simulink model "FULL_CAR_SIM"  (R2025b)
settings: Solver=FixedStepAuto  StartTime=0.0  StopTime=5  FixedStep=dT  RelTol=1e-3
values from neighbouring files (symbols this model uses):
  fc = 50    [FULL_CAR_MODEL.m]
  Fuzzy_Gain = 2300    [FULL_CAR_MODEL.m]
  Kd = 2873    [FULL_CAR_MODEL.m]
  Ki = 250000    [FULL_CAR_MODEL.m]
  Kp = 23750    [FULL_CAR_MODEL.m]
  l1 = 1.2    [FULL_CAR_MODEL.m]
  w1 = 0.7    [FULL_CAR_MODEL.m]
libraries: fuzblock x4, slpidlib x4, simulink x1
settings Model: Creator=andorian  LastModifiedBy=andac

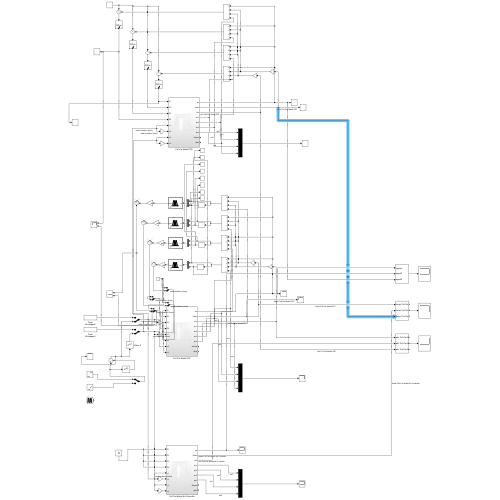
[thumbnail: Simulink's stored preview of the top-level diagram]
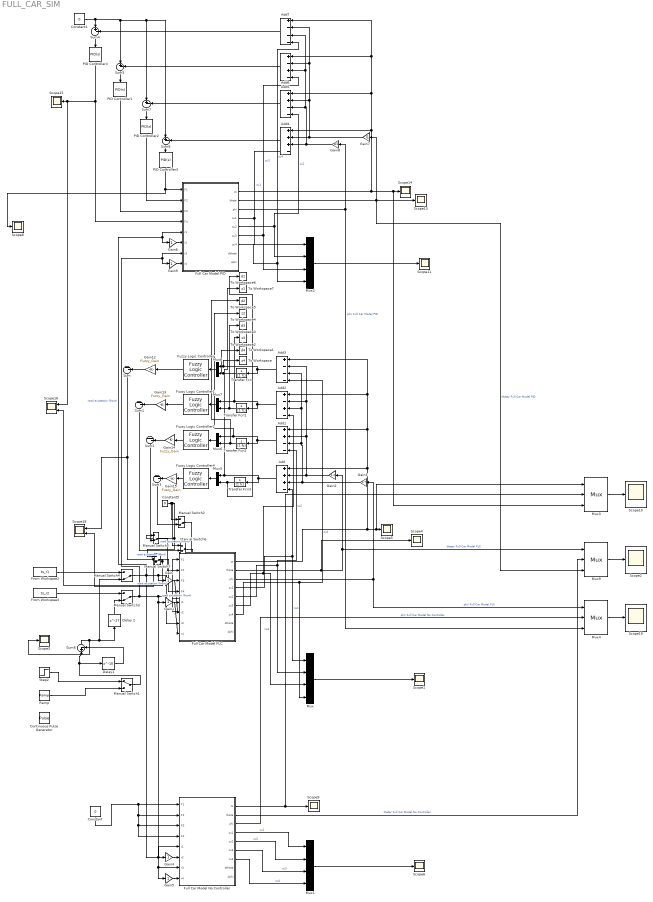
== system FULL_CAR_SIM ==
  Add : Sum  Inputs=+++-
  Add1 : Sum  Inputs=++--
  Add2 : Sum  Inputs=+-+-
  Add3 : Sum  Inputs=+---
  Add4 : Sum  Inputs=+++-
  Add5 : Sum  Inputs=++--
  Add6 : Sum  Inputs=+-+-
  Add7 : Sum  Inputs=+---
  Constant : Constant  Value=0
  Constant1 : Constant  Value=0
  Constant5 : Constant  Value=0
  Continuous Pulse Generator : DiscretePulseGenerator  PulseType=Time based  Period=0.5  PulseWidth=50
  Delay 2 : Delay  DelayLength=27
  Delay1 : Delay  DelayLength=10
  From Workspae2 : FromWorkspace  VariableName=ts_r1
  From Workspae3 : FromWorkspace  VariableName=ts_r2
  Full Car Model FLC : Subsystem
  Full Car Model No Controller : Subsystem
  Full Car Model PID : Subsystem
  Fuzzy Logic Controller{,1..2,4} (4 alike) : fuzblock/Fuzzy Logic  Controller  FIS=susp_fis_cont  OutputSampleNumber=101  DataType=double  UseLookupTable=off  NumBreakpoints=10  FuzzifiedInputs=off  RuleFiringStrengths=off  RuleOutputs=off  AggregatedOutputs=off  SimulateUsing=Interpreted execution  OutOfRangeInputValueMessage=warning  NoRuleFiredMessage=warning  EmptyOutputFuzzySetMessage=warning
  Gain{,1,4..6,9} (6 alike) : Gain
  Gain{12..15} (4 alike) : Gain  Gain=Fuzzy_Gain
  Gain2 : Gain  Gain=1.2
  Gain3 : Gain  Gain=0.7
  Gain7 : Gain  Gain=l1
  Gain8 : Gain  Gain=w1
  Manual Switch1 : ManualSwitch
  Manual Switch{2..7} (6 alike) : ManualSwitch  CurrentSetting=0
  Mux : Mux
  Mux1 : Mux
  Mux2 : Mux
  Mux3 : Mux  Inputs=3
      settings: DisplayOption=signals
  Mux4 : Mux  Inputs=3
      settings: DisplayOption=signals
  Mux{5..8} (4 alike) : Mux  Inputs=2
  Mux9 : Mux  Inputs=3
      settings: DisplayOption=signals
  PID Controller1 : slpidlib/PID Controller  Controller=PID  Form=Parallel  TimeDomain=Continuous-time  UseExternalTs=off  SampleTime=-1  IntegratorMethod=Forward Euler  FilterMethod=Forward Euler  ControllerParametersSource=internal  P=Kp  I=Ki  UseKiTs=off  D=Kd  UseExternalDerivativeSource=off  N=57.4302728612139  UseFilter=on  TunerSelectOption=Transfer Function Based (PID Tuner App)  InitialConditionSource=internal  InitialConditionForIntegrator=0  InitialConditionForFilter=0  DifferentiatorICPrevScaledInput=0  ExternalReset=none  TrackingMode=off  Kt=1  LimitOutput=on  SatLimitsSource=internal  UpperSaturationLimit=2000  LowerSaturationLimit=-2000  LinearizeAsGain=on  AntiWindupMode=back-calculation  Kb=1  LimitIntegrator=off  UpperIntegratorSaturationLimit=inf  LowerIntegratorSaturationLimit=-inf  POutMin=[]  POutMax=[]  IOutMin=[]  IOutMax=[]  DOutMin=[]  DOutMax=[]  NOutMin=[]  NOutMax=[]  SumOutMin=[]  SumOutMax=[]  SaturationOutMin=[]  SaturationOutMax=[]  PParamMin=[]  PParamMax=[]  IParamMin=[]  IParamMax=[]  DParamMin=[]  DParamMax=[]  NParamMin=[]  NParamMax=[]  KbParamMin=[]  KbParamMax=[]  KtParamMin=[]  KtParamMax=[]  KbOutMin=[]  KbOutMax=[]  KtOutMin=[]  KtOutMax=[]  IntegratorOutMin=[]  IntegratorOutMax=[]  FilterOutMin=[]  FilterOutMax=[]  SumI1OutMin=[]  SumI1OutMax=[]  SumI2OutMin=[]  SumI2OutMax=[]  SumI3OutMin=[]  SumI3OutMax=[]  SumI4OutMin=[]  SumI4OutMax=[]  SumDOutMin=[]  SumDOutMax=[]  DifferentiatorOutMin=[]  DifferentiatorOutMax=[]  FilterDiffOutCoefMin=[]  FilterDiffOutCoefMax=[]  ReciprocalOutMin=[]  ReciprocalOutMax=[]  SumDenOutMin=[]  SumDenOutMax=[]  SumNumOutMin=[]  SumNumOutMax=[]  DivideOutMin=[]  DivideOutMax=[]  UdiffTsProdOutMin=[]  UdiffTsProdOutMax=[]  NTsProdOutMin=[]  NTsProdOutMax=[]  UintegralTsProdOutMin=[]  UintegralTsProdOutMax=[]  UngainTsProdOutMin=[]  UngainTsProdOutMax=[]  ClampingZeroOutDataTypeStr=Inherit: Inherit via back propagation  ClampingZeroOutMin=[]  ClampingZeroOutMax=[]  FilterDenConstantOutDataTypeStr=Inherit: Inherit via back propagation  FilterDenConstantOutMin=[]  FilterDenConstantOutMax=[]  PCopyOutDataTypeStr=Inherit: Inherit via back propagation  PCopyOutMin=[]  PCopyOutMax=[]  NCopyOutDataTypeStr=Inherit: Inherit via back propagation  NCopyOutMin=[]  NCopyOutMax=[]  IntegratorContinuousStateAttributes=''  IntegratorStateMustResolveToSignalObject=off  IntegratorRTWStateStorageClass=Auto  FilterContinuousStateAttributes=''  FilterStateMustResolveToSignalObject=off  FilterRTWStateStorageClass=Auto  ParallelPVariant=InternalParameters  IdealPVariant=Disabled  IVariant=InternalParameters  DVariant=InternalParameters  IntegratorVariant=Continuous  SatVariant=Enabled  AWVariant=BackCalculation  PCopyVariant=Disabled  TRVariant=Disabled  FdbkBlocksVariant=Forward  IdealPFdbkVariant=Disabled  SatFdbkVariant=Disabled  DerivativeFilterVariant=ContFilter  NVariant=InternalParameters  NCopyVariant=Disabled  FilterICVariant=InternalICsFilter  IntegratorICVariant=InternalICs  ExternalResetVariant=Disabled  TRSumVariant=Passthrough  SumFdbkVariant=Disabled  SumVariant=Sum_PID  TsampFilterVariant=InternalTs  TsampNgainVariant=Passthrough  TsampIntegralVariant=Disabled_SignalSpec  ExternalSaturationOutDataTypeStr=Inherit: Same as second input  DerivativeSourceVariant=ErrorSignal  PreIntVariant=InternalPreInt
  PID Controller2 : slpidlib/PID Controller  Controller=PID  Form=Parallel  TimeDomain=Continuous-time  UseExternalTs=off  SampleTime=-1  IntegratorMethod=Forward Euler  FilterMethod=Forward Euler  ControllerParametersSource=internal  P=Kp  I=Ki  UseKiTs=off  D=Kd  UseExternalDerivativeSource=off  N=51.5003780888236  UseFilter=on  TunerSelectOption=Transfer Function Based (PID Tuner App)  InitialConditionSource=internal  InitialConditionForIntegrator=0  InitialConditionForFilter=0  DifferentiatorICPrevScaledInput=0  ExternalReset=none  TrackingMode=off  Kt=1  LimitOutput=on  SatLimitsSource=internal  UpperSaturationLimit=2000  LowerSaturationLimit=-2000  LinearizeAsGain=on  AntiWindupMode=back-calculation  Kb=1  LimitIntegrator=off  UpperIntegratorSaturationLimit=inf  LowerIntegratorSaturationLimit=-inf  POutMin=[]  POutMax=[]  IOutMin=[]  IOutMax=[]  DOutMin=[]  DOutMax=[]  NOutMin=[]  NOutMax=[]  SumOutMin=[]  SumOutMax=[]  SaturationOutMin=[]  SaturationOutMax=[]  PParamMin=[]  PParamMax=[]  IParamMin=[]  IParamMax=[]  DParamMin=[]  DParamMax=[]  NParamMin=[]  NParamMax=[]  KbParamMin=[]  KbParamMax=[]  KtParamMin=[]  KtParamMax=[]  KbOutMin=[]  KbOutMax=[]  KtOutMin=[]  KtOutMax=[]  IntegratorOutMin=[]  IntegratorOutMax=[]  FilterOutMin=[]  FilterOutMax=[]  SumI1OutMin=[]  SumI1OutMax=[]  SumI2OutMin=[]  SumI2OutMax=[]  SumI3OutMin=[]  SumI3OutMax=[]  SumI4OutMin=[]  SumI4OutMax=[]  SumDOutMin=[]  SumDOutMax=[]  DifferentiatorOutMin=[]  DifferentiatorOutMax=[]  FilterDiffOutCoefMin=[]  FilterDiffOutCoefMax=[]  ReciprocalOutMin=[]  ReciprocalOutMax=[]  SumDenOutMin=[]  SumDenOutMax=[]  SumNumOutMin=[]  SumNumOutMax=[]  DivideOutMin=[]  DivideOutMax=[]  UdiffTsProdOutMin=[]  UdiffTsProdOutMax=[]  NTsProdOutMin=[]  NTsProdOutMax=[]  UintegralTsProdOutMin=[]  UintegralTsProdOutMax=[]  UngainTsProdOutMin=[]  UngainTsProdOutMax=[]  ClampingZeroOutDataTypeStr=Inherit: Inherit via back propagation  ClampingZeroOutMin=[]  ClampingZeroOutMax=[]  FilterDenConstantOutDataTypeStr=Inherit: Inherit via back propagation  FilterDenConstantOutMin=[]  FilterDenConstantOutMax=[]  PCopyOutDataTypeStr=Inherit: Inherit via back propagation  PCopyOutMin=[]  PCopyOutMax=[]  NCopyOutDataTypeStr=Inherit: Inherit via back propagation  NCopyOutMin=[]  NCopyOutMax=[]  IntegratorContinuousStateAttributes=''  IntegratorStateMustResolveToSignalObject=off  IntegratorRTWStateStorageClass=Auto  FilterContinuousStateAttributes=''  FilterStateMustResolveToSignalObject=off  FilterRTWStateStorageClass=Auto  ParallelPVariant=InternalParameters  IdealPVariant=Disabled  IVariant=InternalParameters  DVariant=InternalParameters  IntegratorVariant=Continuous  SatVariant=Enabled  AWVariant=BackCalculation  PCopyVariant=Disabled  TRVariant=Disabled  FdbkBlocksVariant=Forward  IdealPFdbkVariant=Disabled  SatFdbkVariant=Disabled  DerivativeFilterVariant=ContFilter  NVariant=InternalParameters  NCopyVariant=Disabled  FilterICVariant=InternalICsFilter  IntegratorICVariant=InternalICs  ExternalResetVariant=Disabled  TRSumVariant=Passthrough  SumFdbkVariant=Disabled  SumVariant=Sum_PID  TsampFilterVariant=InternalTs  TsampNgainVariant=Passthrough  TsampIntegralVariant=Disabled_SignalSpec  ExternalSaturationOutDataTypeStr=Inherit: Same as second input  DerivativeSourceVariant=ErrorSignal  PreIntVariant=InternalPreInt
  PID Controller3 : slpidlib/PID Controller  Controller=PID  Form=Parallel  TimeDomain=Continuous-time  UseExternalTs=off  SampleTime=-1  IntegratorMethod=Forward Euler  FilterMethod=Forward Euler  ControllerParametersSource=internal  P=Kp  I=Ki  UseKiTs=off  D=Kd  UseExternalDerivativeSource=off  N=52.4135371297366  UseFilter=on  TunerSelectOption=Transfer Function Based (PID Tuner App)  InitialConditionSource=internal  InitialConditionForIntegrator=0  InitialConditionForFilter=0  DifferentiatorICPrevScaledInput=0  ExternalReset=none  TrackingMode=off  Kt=1  LimitOutput=on  SatLimitsSource=internal  UpperSaturationLimit=2000  LowerSaturationLimit=-2000  LinearizeAsGain=on  AntiWindupMode=back-calculation  Kb=1  LimitIntegrator=off  UpperIntegratorSaturationLimit=inf  LowerIntegratorSaturationLimit=-inf  POutMin=[]  POutMax=[]  IOutMin=[]  IOutMax=[]  DOutMin=[]  DOutMax=[]  NOutMin=[]  NOutMax=[]  SumOutMin=[]  SumOutMax=[]  SaturationOutMin=[]  SaturationOutMax=[]  PParamMin=[]  PParamMax=[]  IParamMin=[]  IParamMax=[]  DParamMin=[]  DParamMax=[]  NParamMin=[]  NParamMax=[]  KbParamMin=[]  KbParamMax=[]  KtParamMin=[]  KtParamMax=[]  KbOutMin=[]  KbOutMax=[]  KtOutMin=[]  KtOutMax=[]  IntegratorOutMin=[]  IntegratorOutMax=[]  FilterOutMin=[]  FilterOutMax=[]  SumI1OutMin=[]  SumI1OutMax=[]  SumI2OutMin=[]  SumI2OutMax=[]  SumI3OutMin=[]  SumI3OutMax=[]  SumI4OutMin=[]  SumI4OutMax=[]  SumDOutMin=[]  SumDOutMax=[]  DifferentiatorOutMin=[]  DifferentiatorOutMax=[]  FilterDiffOutCoefMin=[]  FilterDiffOutCoefMax=[]  ReciprocalOutMin=[]  ReciprocalOutMax=[]  SumDenOutMin=[]  SumDenOutMax=[]  SumNumOutMin=[]  SumNumOutMax=[]  DivideOutMin=[]  DivideOutMax=[]  UdiffTsProdOutMin=[]  UdiffTsProdOutMax=[]  NTsProdOutMin=[]  NTsProdOutMax=[]  UintegralTsProdOutMin=[]  UintegralTsProdOutMax=[]  UngainTsProdOutMin=[]  UngainTsProdOutMax=[]  ClampingZeroOutDataTypeStr=Inherit: Inherit via back propagation  ClampingZeroOutMin=[]  ClampingZeroOutMax=[]  FilterDenConstantOutDataTypeStr=Inherit: Inherit via back propagation  FilterDenConstantOutMin=[]  FilterDenConstantOutMax=[]  PCopyOutDataTypeStr=Inherit: Inherit via back propagation  PCopyOutMin=[]  PCopyOutMax=[]  NCopyOutDataTypeStr=Inherit: Inherit via back propagation  NCopyOutMin=[]  NCopyOutMax=[]  IntegratorContinuousStateAttributes=''  IntegratorStateMustResolveToSignalObject=off  IntegratorRTWStateStorageClass=Auto  FilterContinuousStateAttributes=''  FilterStateMustResolveToSignalObject=off  FilterRTWStateStorageClass=Auto  ParallelPVariant=InternalParameters  IdealPVariant=Disabled  IVariant=InternalParameters  DVariant=InternalParameters  IntegratorVariant=Continuous  SatVariant=Enabled  AWVariant=BackCalculation  PCopyVariant=Disabled  TRVariant=Disabled  FdbkBlocksVariant=Forward  IdealPFdbkVariant=Disabled  SatFdbkVariant=Disabled  DerivativeFilterVariant=ContFilter  NVariant=InternalParameters  NCopyVariant=Disabled  FilterICVariant=InternalICsFilter  IntegratorICVariant=InternalICs  ExternalResetVariant=Disabled  TRSumVariant=Passthrough  SumFdbkVariant=Disabled  SumVariant=Sum_PID  TsampFilterVariant=InternalTs  TsampNgainVariant=Passthrough  TsampIntegralVariant=Disabled_SignalSpec  ExternalSaturationOutDataTypeStr=Inherit: Same as second input  DerivativeSourceVariant=ErrorSignal  PreIntVariant=InternalPreInt
  PID Controller4 : slpidlib/PID Controller  Controller=PID  Form=Parallel  TimeDomain=Continuous-time  UseExternalTs=off  SampleTime=-1  IntegratorMethod=Forward Euler  FilterMethod=Forward Euler  ControllerParametersSource=internal  P=Kp  I=Ki  UseKiTs=off  D=Kd  UseExternalDerivativeSource=off  N=50.65220146303482  UseFilter=on  TunerSelectOption=Transfer Function Based (PID Tuner App)  InitialConditionSource=internal  InitialConditionForIntegrator=0  InitialConditionForFilter=0  DifferentiatorICPrevScaledInput=0  ExternalReset=none  TrackingMode=off  Kt=1  LimitOutput=on  SatLimitsSource=internal  UpperSaturationLimit=2000  LowerSaturationLimit=-2000  LinearizeAsGain=on  AntiWindupMode=back-calculation  Kb=1  LimitIntegrator=off  UpperIntegratorSaturationLimit=inf  LowerIntegratorSaturationLimit=-inf  POutMin=[]  POutMax=[]  IOutMin=[]  IOutMax=[]  DOutMin=[]  DOutMax=[]  NOutMin=[]  NOutMax=[]  SumOutMin=[]  SumOutMax=[]  SaturationOutMin=[]  SaturationOutMax=[]  PParamMin=[]  PParamMax=[]  IParamMin=[]  IParamMax=[]  DParamMin=[]  DParamMax=[]  NParamMin=[]  NParamMax=[]  KbParamMin=[]  KbParamMax=[]  KtParamMin=[]  KtParamMax=[]  KbOutMin=[]  KbOutMax=[]  KtOutMin=[]  KtOutMax=[]  IntegratorOutMin=[]  IntegratorOutMax=[]  FilterOutMin=[]  FilterOutMax=[]  SumI1OutMin=[]  SumI1OutMax=[]  SumI2OutMin=[]  SumI2OutMax=[]  SumI3OutMin=[]  SumI3OutMax=[]  SumI4OutMin=[]  SumI4OutMax=[]  SumDOutMin=[]  SumDOutMax=[]  DifferentiatorOutMin=[]  DifferentiatorOutMax=[]  FilterDiffOutCoefMin=[]  FilterDiffOutCoefMax=[]  ReciprocalOutMin=[]  ReciprocalOutMax=[]  SumDenOutMin=[]  SumDenOutMax=[]  SumNumOutMin=[]  SumNumOutMax=[]  DivideOutMin=[]  DivideOutMax=[]  UdiffTsProdOutMin=[]  UdiffTsProdOutMax=[]  NTsProdOutMin=[]  NTsProdOutMax=[]  UintegralTsProdOutMin=[]  UintegralTsProdOutMax=[]  UngainTsProdOutMin=[]  UngainTsProdOutMax=[]  ClampingZeroOutDataTypeStr=Inherit: Inherit via back propagation  ClampingZeroOutMin=[]  ClampingZeroOutMax=[]  FilterDenConstantOutDataTypeStr=Inherit: Inherit via back propagation  FilterDenConstantOutMin=[]  FilterDenConstantOutMax=[]  PCopyOutDataTypeStr=Inherit: Inherit via back propagation  PCopyOutMin=[]  PCopyOutMax=[]  NCopyOutDataTypeStr=Inherit: Inherit via back propagation  NCopyOutMin=[]  NCopyOutMax=[]  IntegratorContinuousStateAttributes=''  IntegratorStateMustResolveToSignalObject=off  IntegratorRTWStateStorageClass=Auto  FilterContinuousStateAttributes=''  FilterStateMustResolveToSignalObject=off  FilterRTWStateStorageClass=Auto  ParallelPVariant=InternalParameters  IdealPVariant=Disabled  IVariant=InternalParameters  DVariant=InternalParameters  IntegratorVariant=Continuous  SatVariant=Enabled  AWVariant=BackCalculation  PCopyVariant=Disabled  TRVariant=Disabled  FdbkBlocksVariant=Forward  IdealPFdbkVariant=Disabled  SatFdbkVariant=Disabled  DerivativeFilterVariant=ContFilter  NVariant=InternalParameters  NCopyVariant=Disabled  FilterICVariant=InternalICsFilter  IntegratorICVariant=InternalICs  ExternalResetVariant=Disabled  TRSumVariant=Passthrough  SumFdbkVariant=Disabled  SumVariant=Sum_PID  TsampFilterVariant=InternalTs  TsampNgainVariant=Passthrough  TsampIntegralVariant=Disabled_SignalSpec  ExternalSaturationOutDataTypeStr=Inherit: Same as second input  DerivativeSourceVariant=ErrorSignal  PreIntVariant=InternalPreInt
  Ramp : simulink/Sources/Ramp  slope=1  start=0  InitialOutput=0
  Scope{1..6,8..11,13..15,19} (14 alike) : Scope
      Scope1 settings: ActiveDisplayYMinimum=-0.0297  ActiveDisplayYMaximum=0.0637
      Scope10 settings: ActiveDisplayYMinimum=-0.062727148676568811  ActiveDisplayYMaximum=0.13515814704909826  DataLoggingVariableName=ScopeData9
      Scope11 settings: ActiveDisplayYMinimum=-0.02379  ActiveDisplayYMaximum=0.02112  DataLoggingVariableName=ScopeData10
      Scope13 settings: ActiveDisplayYMinimum=-1  ActiveDisplayYMaximum=1  DataLoggingVariableName=ScopeData12
      Scope14 settings: ActiveDisplayYMinimum=-0.00675  ActiveDisplayYMaximum=0.01662  DataLoggingVariableName=ScopeData13
      Scope15 settings: ActiveDisplayYMinimum=-0.01471  ActiveDisplayYMaximum=0.0084  DataLoggingVariableName=ScopeData2
      Scope19 settings: ActiveDisplayYMinimum=-0.00025045373709102042  ActiveDisplayYMaximum=0.00024417813844507355
      Scope2 settings: ActiveDisplayYMinimum=-0.039144903517554647  ActiveDisplayYMaximum=0.045294756632955478  DataLoggingVariableName=ScopeData2
      Scope3 settings: ActiveDisplayYMinimum=-1.5419809912420392  ActiveDisplayYMaximum=1.3520815087579612
      Scope4 settings: ActiveDisplayYMinimum=-0.00958  ActiveDisplayYMaximum=0.00964  DataLoggingVariableName=ScopeData3
      Scope5 settings: ActiveDisplayYMinimum=-0.00675  ActiveDisplayYMaximum=0.01662  DataLoggingVariableName=ScopeData4
      Scope6 settings: ActiveDisplayYMinimum=-0.45427  ActiveDisplayYMaximum=0.44698  DataLoggingVariableName=ScopeData5
      Scope8 settings: ActiveDisplayYMinimum=-7476.042628084072  ActiveDisplayYMaximum=8515.0328459762477  DataLoggingVariableName=ScopeData6
      Scope9 settings: ActiveDisplayYMinimum=-0.00675  ActiveDisplayYMaximum=0.01662  DataLoggingVariableName=ScopeData8
  Scope16 : Scope  NumInputPorts=2
      settings: ActiveDisplayYMinimum=-0.01508  ActiveDisplayYMaximum=0.01168  DataLoggingVariableName=ScopeData3
  Scope18 : Scope  NumInputPorts=2
      settings: ActiveDisplayYMinimum=-0.00554  ActiveDisplayYMaximum=0.00333
  Step2 : Step  Time=2  Before=1  SampleTime=0
  Sum{,1..3} (4 alike) : Sum  Inputs=|---
  Sum{4..8} (5 alike) : Sum  Inputs=|+-
  To Workspace : ToWorkspace  VariableName=z4  SampleTime=-1
      settings: Save2DSignal=2-D array (concatenate along first dimension)
  To Workspace1 : ToWorkspace  VariableName=d4  SampleTime=-1
      settings: Save2DSignal=2-D array (concatenate along first dimension)
  To Workspace2 : ToWorkspace  VariableName=z3  SampleTime=-1
      settings: Save2DSignal=2-D array (concatenate along first dimension)
  To Workspace3 : ToWorkspace  VariableName=d3  SampleTime=-1
      settings: Save2DSignal=2-D array (concatenate along first dimension)
  To Workspace4 : ToWorkspace  VariableName=z2  SampleTime=-1
      settings: Save2DSignal=2-D array (concatenate along first dimension)
  To Workspace5 : ToWorkspace  VariableName=d2  SampleTime=-1
      settings: Save2DSignal=2-D array (concatenate along first dimension)
  To Workspace6 : ToWorkspace  VariableName=d1  SampleTime=-1
      settings: Save2DSignal=2-D array (concatenate along first dimension)
  To Workspace7 : ToWorkspace  VariableName=z1  SampleTime=-1
      settings: Save2DSignal=2-D array (concatenate along first dimension)
  Transfer Fcn{,1..3} (4 alike) : TransferFcn  Numerator=[1 0]  Denominator=[1 fc]
  wires:
  Full Car Model FLC/1(zs) -> Add/1, Add3/1, Add2/1, Add1/1, Mux3/1, Scope5/1
  Full Car Model FLC/3(phi) -> Mux4/1, Gain3/1  "phi/ Full Car Model FLC"
  Full Car Model FLC/4(zu1) -> Mux/1, Add/4  "zu1"
  Full Car Model FLC/5(zu2) -> Add1/4, Mux/2  "zu2"
  Full Car Model FLC/6(zu3) -> Add2/4, Mux/3  "zu3"
  Full Car Model FLC/7(zu4) -> Add3/4, Mux/4  "zu4"
  Mux/1 -> Scope1/1
  Delay1/1 -> Sum6/2
  From Workspae2/1 -> Manual Switch4/1
  Step2/1 -> Manual Switch1/1
  Delay 2/1 -> Manual Switch3/2
  Manual Switch1/1 -> Delay1/1, Sum6/1
  From Workspae3/1 -> Manual Switch3/1
  Sum6/1 -> Scope3/1, Delay 2/1, Manual Switch4/2
  Full Car Model FLC/2(theta) -> Gain2/1, Mux9/1, Scope4/1  "theta/ Full Car Model FLC"
  Gain/1 -> Full Car Model FLC/6(r2)
  Gain1/1 -> Full Car Model FLC/8(r4)
  Gain2/1 -> Add/2, Add1/2, Add3/2, Add2/2
  Gain3/1 -> Add/3, Add3/3, Add2/3, Add1/3
  Fuzzy Logic Controller1/1 -> Gain13/1
  Full Car Model No Controller/2(theta) -> Mux9/2  "theta/ Full Car Model No Controller"
  Manual Switch4/1 -> Gain6/1, Full Car Model PID/5(r1), Full Car Model No Controller/5(r1), Gain4/1, Gain/1, Full Car Model FLC/5(r1)  "road excitation (front)"
  Gain4/1 -> Full Car Model No Controller/6(r2)
  Full Car Model No Controller/5(zu2) -> Mux1/2  "zu2"
  Full Car Model No Controller/6(zu3) -> Mux1/3  "zu3"
  Full Car Model No Controller/4(zu1) -> Mux1/1  "zu1"
  Gain5/1 -> Full Car Model No Controller/8(r4)
  Full Car Model No Controller/7(zu4) -> Mux1/4  "zu4"
  Full Car Model No Controller/1(zs) -> Mux3/2, Scope9/1
  Mux1/1 -> Scope6/1
  Constant/1 -> Full Car Model No Controller/1(F1), Full Car Model No Controller/4(F4), Full Car Model No Controller/3(F3), Full Car Model No Controller/2(F2)
  Gain8/1 -> Add4/3, Add7/3, Add6/3, Add5/3
  Gain7/1 -> Add4/2, Add5/2, Add6/2, Add7/2
  Full Car Model PID/2(theta) -> Mux9/3, Scope13/1, Gain7/1  "theta/ Full Car Model PID"
  Gain6/1 -> Full Car Model PID/6(r2)
  Manual Switch3/1 -> Gain9/1, Full Car Model PID/7(r3), Gain5/1, Full Car Model No Controller/7(r3), Gain1/1, Full Car Model FLC/7(r3)
  Full Car Model PID/5(zu2) -> Add5/4, Mux2/2  "zu2"
  Full Car Model PID/3(phi) -> Gain8/1, Mux4/3  "phi/ Full Car Model PID"
  Full Car Model PID/6(zu3) -> Add6/4, Mux2/3  "zu3"
  Mux2/1 -> Scope11/1
  Full Car Model PID/4(zu1) -> Mux2/1, Add4/4  "zu1"
  Full Car Model PID/7(zu4) -> Add7/4, Mux2/4  "zu4"
  Full Car Model PID/1(zs) -> Add4/1, Add7/1, Add6/1, Add5/1, Mux3/3, Scope14/1
  Gain9/1 -> Full Car Model PID/8(r4)
  Add7/1 -> Sum4/2
  Sum4/1 -> PID Controller4/1
  Add6/1 -> Sum5/2
  Sum5/1 -> PID Controller1/1
  Sum7/1 -> PID Controller2/1
  Sum8/1 -> PID Controller3/1
  Mux3/1 -> Scope10/1
  Mux5/1 -> Fuzzy Logic Controller4/1
  Mux6/1 -> Fuzzy Logic Controller2/1
  Mux7/1 -> Fuzzy Logic Controller1/1
  Mux8/1 -> Fuzzy Logic Controller/1
  Transfer Fcn/1 -> To Workspace1/1, Mux8/2
  Add3/1 -> Transfer Fcn/1, To Workspace/1, Mux8/1
  Sum3/1 -> Manual Switch2/2
  Sum2/1 -> Manual Switch5/2
  Sum1/1 -> Manual Switch6/2
  Sum/1 -> Scope18/2, Manual Switch7/2, Scope16/2, Scope18/1
  Ramp/1 -> Manual Switch1/2
  Fuzzy Logic Controller/1 -> Gain12/1
  Fuzzy Logic Controller2/1 -> Gain14/1
  Fuzzy Logic Controller4/1 -> Gain15/1
  Gain12/1 -> Sum/3
  Gain13/1 -> Sum1/3
  Gain14/1 -> Sum2/3
  Gain15/1 -> Sum3/3
  Add2/1 -> Transfer Fcn1/1, Mux7/1, To Workspace2/1
  Transfer Fcn1/1 -> To Workspace3/1, Mux7/2
  Add1/1 -> Transfer Fcn2/1, Mux6/1, To Workspace4/1
  Transfer Fcn2/1 -> To Workspace5/1, Mux6/2
  Transfer Fcn3/1 -> To Workspace6/1, Mux5/2
  Add/1 -> Transfer Fcn3/1, Mux5/1, To Workspace7/1
  Manual Switch2/1 -> Full Car Model FLC/1(F1)  "road excitation (front)"
  Manual Switch5/1 -> Full Car Model FLC/2(F2)  "road excitation (front)"
  Manual Switch6/1 -> Full Car Model FLC/3(F3)  "road excitation (front)"
  Manual Switch7/1 -> Full Car Model FLC/4(F4)  "road excitation (front)"
  Constant5/1 -> Manual Switch7/1, Manual Switch5/1, Manual Switch6/1, Manual Switch2/1
  Mux4/1 -> Scope19/1
  Full Car Model No Controller/3(phi) -> Mux4/2  "phi/ Full Car Model No Controller"
  Mux9/1 -> Scope2/1
  Add5/1 -> Sum7/2
  Add4/1 -> Sum8/2
  PID Controller3/1 -> Full Car Model PID/1(F1), Scope8/1
  PID Controller2/1 -> Full Car Model PID/2(F2)
  PID Controller1/1 -> Full Car Model PID/3(F3)
  PID Controller4/1 -> Full Car Model PID/4(F4), Scope16/1, Scope15/1
  Constant1/1 -> Sum8/1, Sum7/1, Sum5/1, Sum4/1

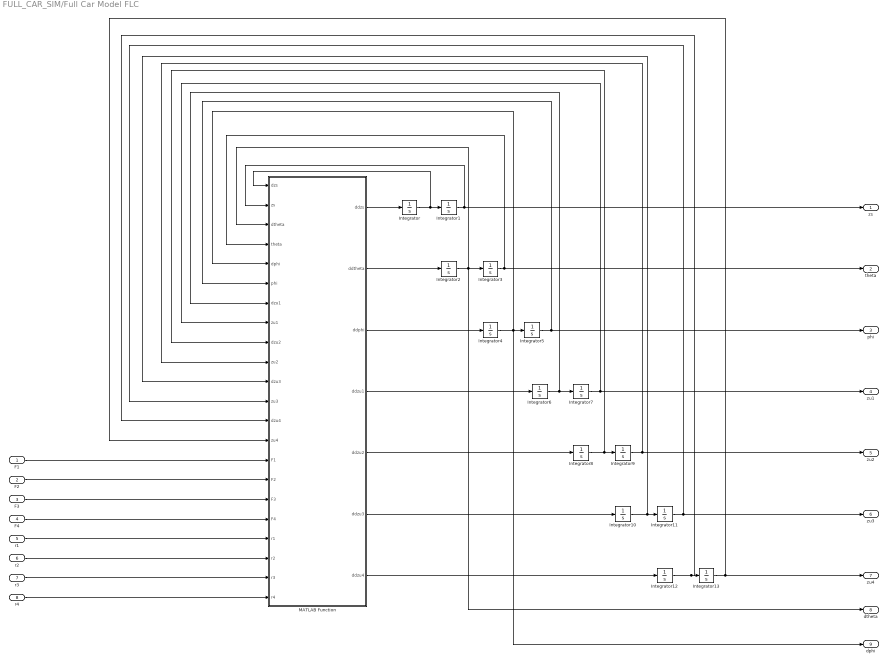
== system FULL_CAR_SIM/Full Car Model FLC ==
  F1 : Inport
  F2 : Inport  Port=2
  F3 : Inport  Port=3
  F4 : Inport  Port=4
  r1 : Inport  Port=5
  r2 : Inport  Port=6
  r3 : Inport  Port=7
  r4 : Inport  Port=8
  Integrator{,1..13} (14 alike) : Integrator
  MATLAB Function : MATLAB Function  TreatAsAtomicUnit=on
  zs : Outport
  theta : Outport  Port=2
  phi : Outport  Port=3
  zu1 : Outport  Port=4
  zu2 : Outport  Port=5
  zu3 : Outport  Port=6
  zu4 : Outport  Port=7
  dtheta : Outport  Port=8
  dphi : Outport  Port=9
  wires:
  Integrator4/1 -> dphi/1, Integrator5/1, MATLAB Function/5(dphi)
  MATLAB Function/2(ddtheta) -> Integrator2/1
  Integrator9/1 -> zu2/1, MATLAB Function/10(zu2)
  Integrator2/1 -> dtheta/1, Integrator3/1, MATLAB Function/3(dtheta)
  MATLAB Function/7(ddzu4) -> Integrator12/1
  Integrator10/1 -> MATLAB Function/11(dzu3), Integrator11/1
  Integrator1/1 -> zs/1, MATLAB Function/2(zs)
  F4/1 -> MATLAB Function/18(F4)
  MATLAB Function/1(ddzs) -> Integrator/1
  Integrator13/1 -> zu4/1, MATLAB Function/14(zu4)
  r1/1 -> MATLAB Function/19(r1)
  Integrator5/1 -> phi/1, MATLAB Function/6(phi)
  Integrator12/1 -> MATLAB Function/13(dzu4), Integrator13/1
  MATLAB Function/3(ddphi) -> Integrator4/1
  Integrator7/1 -> zu1/1, MATLAB Function/8(zu1)
  Integrator/1 -> MATLAB Function/1(dzs), Integrator1/1
  MATLAB Function/5(ddzu2) -> Integrator8/1
  r4/1 -> MATLAB Function/22(r4)
  MATLAB Function/4(ddzu1) -> Integrator6/1
  Integrator6/1 -> MATLAB Function/7(dzu1), Integrator7/1
  Integrator3/1 -> theta/1, MATLAB Function/4(theta)
  F2/1 -> MATLAB Function/16(F2)
  F1/1 -> MATLAB Function/15(F1)
  F3/1 -> MATLAB Function/17(F3)
  Integrator11/1 -> zu3/1, MATLAB Function/12(zu3)
  r3/1 -> MATLAB Function/21(r3)
  r2/1 -> MATLAB Function/20(r2)
  Integrator8/1 -> MATLAB Function/9(dzu2), Integrator9/1
  MATLAB Function/6(ddzu3) -> Integrator10/1

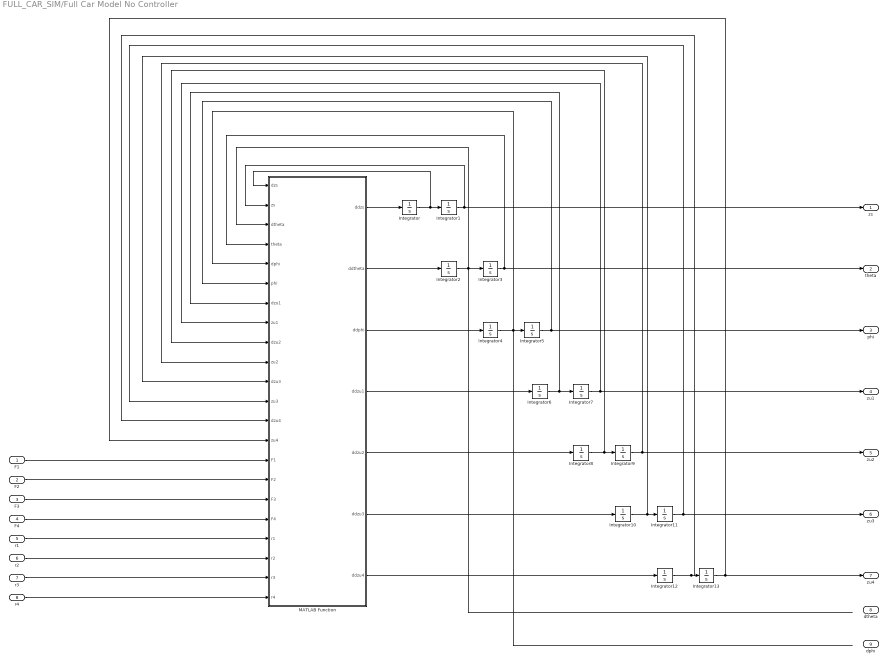
== system FULL_CAR_SIM/Full Car Model No Controller ==
  F1 : Inport
  F2 : Inport  Port=2
  F3 : Inport  Port=3
  F4 : Inport  Port=4
  r1 : Inport  Port=5
  r2 : Inport  Port=6
  r3 : Inport  Port=7
  r4 : Inport  Port=8
  Integrator{,1..13} (14 alike) : Integrator
  MATLAB Function : MATLAB Function  TreatAsAtomicUnit=on
  zs : Outport
  theta : Outport  Port=2
  phi : Outport  Port=3
  zu1 : Outport  Port=4
  zu2 : Outport  Port=5
  zu3 : Outport  Port=6
  zu4 : Outport  Port=7
  dtheta : Outport  Port=8
  dphi : Outport  Port=9
  wires:
  Integrator4/1 -> Integrator5/1, MATLAB Function/5(dphi)
  MATLAB Function/2(ddtheta) -> Integrator2/1
  Integrator9/1 -> zu2/1, MATLAB Function/10(zu2)
  Integrator2/1 -> Integrator3/1, MATLAB Function/3(dtheta)
  MATLAB Function/7(ddzu4) -> Integrator12/1
  Integrator10/1 -> MATLAB Function/11(dzu3), Integrator11/1
  Integrator1/1 -> zs/1, MATLAB Function/2(zs)
  F4/1 -> MATLAB Function/18(F4)
  MATLAB Function/1(ddzs) -> Integrator/1
  Integrator13/1 -> zu4/1, MATLAB Function/14(zu4)
  r1/1 -> MATLAB Function/19(r1)
  Integrator5/1 -> phi/1, MATLAB Function/6(phi)
  Integrator12/1 -> MATLAB Function/13(dzu4), Integrator13/1
  MATLAB Function/3(ddphi) -> Integrator4/1
  Integrator7/1 -> zu1/1, MATLAB Function/8(zu1)
  Integrator/1 -> MATLAB Function/1(dzs), Integrator1/1
  MATLAB Function/5(ddzu2) -> Integrator8/1
  r4/1 -> MATLAB Function/22(r4)
  MATLAB Function/4(ddzu1) -> Integrator6/1
  Integrator6/1 -> MATLAB Function/7(dzu1), Integrator7/1
  Integrator3/1 -> theta/1, MATLAB Function/4(theta)
  F2/1 -> MATLAB Function/16(F2)
  F1/1 -> MATLAB Function/15(F1)
  F3/1 -> MATLAB Function/17(F3)
  Integrator11/1 -> zu3/1, MATLAB Function/12(zu3)
  r3/1 -> MATLAB Function/21(r3)
  r2/1 -> MATLAB Function/20(r2)
  Integrator8/1 -> MATLAB Function/9(dzu2), Integrator9/1
  MATLAB Function/6(ddzu3) -> Integrator10/1

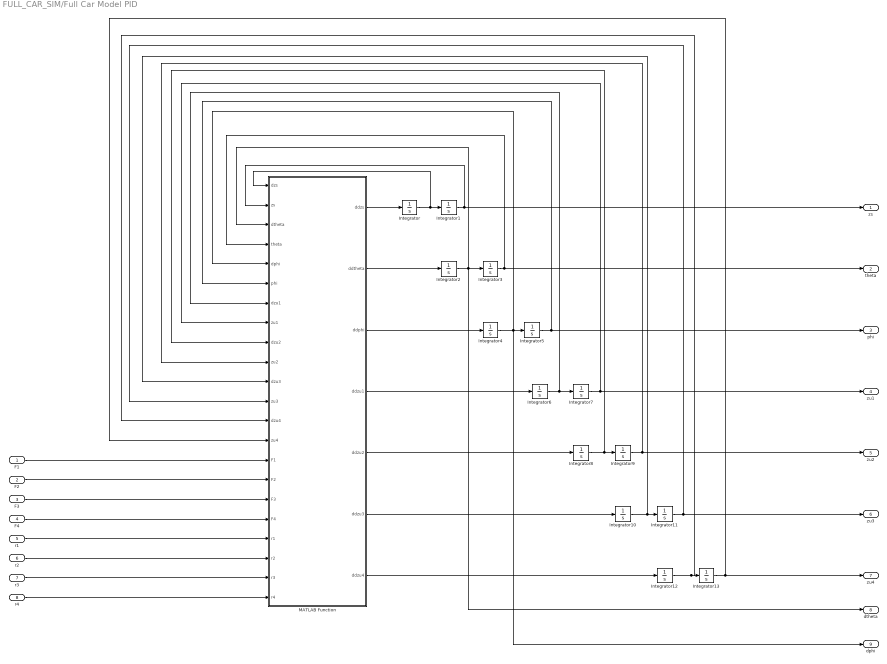
== system FULL_CAR_SIM/Full Car Model PID ==
  F1 : Inport
  F2 : Inport  Port=2
  F3 : Inport  Port=3
  F4 : Inport  Port=4
  r1 : Inport  Port=5
  r2 : Inport  Port=6
  r3 : Inport  Port=7
  r4 : Inport  Port=8
  Integrator{,1..13} (14 alike) : Integrator
  MATLAB Function : MATLAB Function  TreatAsAtomicUnit=on
  zs : Outport
  theta : Outport  Port=2
  phi : Outport  Port=3
  zu1 : Outport  Port=4
  zu2 : Outport  Port=5
  zu3 : Outport  Port=6
  zu4 : Outport  Port=7
  dtheta : Outport  Port=8
  dphi : Outport  Port=9
  wires:
  Integrator4/1 -> dphi/1, Integrator5/1, MATLAB Function/5(dphi)
  MATLAB Function/2(ddtheta) -> Integrator2/1
  Integrator9/1 -> zu2/1, MATLAB Function/10(zu2)
  Integrator2/1 -> dtheta/1, Integrator3/1, MATLAB Function/3(dtheta)
  MATLAB Function/7(ddzu4) -> Integrator12/1
  Integrator10/1 -> MATLAB Function/11(dzu3), Integrator11/1
  Integrator1/1 -> zs/1, MATLAB Function/2(zs)
  F4/1 -> MATLAB Function/18(F4)
  MATLAB Function/1(ddzs) -> Integrator/1
  Integrator13/1 -> zu4/1, MATLAB Function/14(zu4)
  r1/1 -> MATLAB Function/19(r1)
  Integrator5/1 -> phi/1, MATLAB Function/6(phi)
  Integrator12/1 -> MATLAB Function/13(dzu4), Integrator13/1
  MATLAB Function/3(ddphi) -> Integrator4/1
  Integrator7/1 -> zu1/1, MATLAB Function/8(zu1)
  Integrator/1 -> MATLAB Function/1(dzs), Integrator1/1
  MATLAB Function/5(ddzu2) -> Integrator8/1
  r4/1 -> MATLAB Function/22(r4)
  MATLAB Function/4(ddzu1) -> Integrator6/1
  Integrator6/1 -> MATLAB Function/7(dzu1), Integrator7/1
  Integrator3/1 -> theta/1, MATLAB Function/4(theta)
  F2/1 -> MATLAB Function/16(F2)
  F1/1 -> MATLAB Function/15(F1)
  F3/1 -> MATLAB Function/17(F3)
  Integrator11/1 -> zu3/1, MATLAB Function/12(zu3)
  r3/1 -> MATLAB Function/21(r3)
  r2/1 -> MATLAB Function/20(r2)
  Integrator8/1 -> MATLAB Function/9(dzu2), Integrator9/1
  MATLAB Function/6(ddzu3) -> Integrator10/1

== matlab function FULL_CAR_SIM/Full Car Model PID/MATLAB Function ==
  data: dzs input; zs input; dtheta input; ddzs output; theta input; dphi input; phi input; dzu1 input; zu1 input; dzu2 input; zu2 input; dzu3 input; zu3 input; dzu4 input; zu4 input; F1 input; F2 input; F3 input; F4 input; r1 input; r2 input; ddtheta output; ddphi output; ddzu1 output; ddzu2 output; ddzu3 output; ddzu4 output; r3 input; r4 input
function [ddzs, ddtheta, ddphi, ddzu1, ddzu2, ddzu3, ddzu4] = suspension_dynamics(dzs, zs, dtheta, theta, dphi, phi, dzu1, zu1, dzu2, zu2,  dzu3, zu3, dzu4, zu4, F1, F2, F3, F4,r1, r2, r3, r4)

ddzs = F1/1000 + F2/1000 + F3/1000 + F4/1000 + (2253*dtheta)/2500 - (751*dzs)/125 + (751*dzu1)/500 + (751*dzu2)/500 + (751*dzu3)/500 + (751*dzu4)/500 + 18*theta - 120*zs + 30*zu1 + 30*zu2 + 30*zu3 + 30*zu4;
 
 
ddtheta = F1/1000 + F2/1000 - F3/800 - F4/800 - (92373*dtheta)/10000 + (751*dzs)/1000 + (751*dzu1)/500 + (751*dzu2)/500 - (751*dzu3)/400 - (751*dzu4)/400 - (369*theta)/2 + 15*zs + 30*zu1 + 30*zu2 - (75*zu3)/2 - (75*zu4)/2;
 
 
ddphi = (7*F1)/12000 - (7*F2)/12000 + (7*F3)/12000 - (7*F4)/12000 - (36799*dphi)/15000 + (5257*dzu1)/6000 - (5257*dzu2)/6000 + (5257*dzu3)/6000 - (5257*dzu4)/6000 - 49*phi + (35*zu1)/2 - (35*zu2)/2 + (35*zu3)/2 - (35*zu4)/2;
 
 
ddzu1 = (751*dphi)/50 - F1/70 + (4506*dtheta)/175 + (751*dzs)/35 - (751*dzu1)/35 + 300*phi + (20000*r1)/7 + (3600*theta)/7 + (3000*zs)/7 - (23000*zu1)/7;
 
 
ddzu2 = (4506*dtheta)/175 - (751*dphi)/50 - F2/70 + (751*dzs)/35 - (751*dzu2)/35 - 300*phi + (20000*r2)/7 + (3600*theta)/7 + (3000*zs)/7 - (23000*zu2)/7;
 
 
ddzu3 = (751*dphi)/50 - F3/70 - (2253*dtheta)/70 + (751*dzs)/35 - (751*dzu3)/35 + 300*phi + (20000*r3)/7 - (4500*theta)/7 + (3000*zs)/7 - (23000*zu3)/7;
 
 
ddzu4 = (751*dzs)/35 - (751*dphi)/50 - (2253*dtheta)/70 - F4/70 - (751*dzu4)/35 - 300*phi + (20000*r4)/7 - (4500*theta)/7 + (3000*zs)/7 - (23000*zu4)/7;
end

== matlab function FULL_CAR_SIM/Full Car Model No Controller/MATLAB Function ==
  data: dzs input; zs input; dtheta input; ddzs output; theta input; dphi input; phi input; dzu1 input; zu1 input; dzu2 input; zu2 input; dzu3 input; zu3 input; dzu4 input; zu4 input; F1 input; F2 input; F3 input; F4 input; r1 input; r2 input; ddtheta output; ddphi output; ddzu1 output; ddzu2 output; ddzu3 output; ddzu4 output; r3 input; r4 input
function [ddzs, ddtheta, ddphi, ddzu1, ddzu2, ddzu3, ddzu4] = suspension_dynamics(dzs, zs, dtheta, theta, dphi, phi, dzu1, zu1, dzu2, zu2,  dzu3, zu3, dzu4, zu4, F1, F2, F3, F4,r1, r2, r3, r4)

ddzs = F1/1000 + F2/1000 + F3/1000 + F4/1000 + (2253*dtheta)/2500 - (751*dzs)/125 + (751*dzu1)/500 + (751*dzu2)/500 + (751*dzu3)/500 + (751*dzu4)/500 + 18*theta - 120*zs + 30*zu1 + 30*zu2 + 30*zu3 + 30*zu4;
 
 
ddtheta = F1/1000 + F2/1000 - F3/800 - F4/800 - (92373*dtheta)/10000 + (751*dzs)/1000 + (751*dzu1)/500 + (751*dzu2)/500 - (751*dzu3)/400 - (751*dzu4)/400 - (369*theta)/2 + 15*zs + 30*zu1 + 30*zu2 - (75*zu3)/2 - (75*zu4)/2;
 
 
ddphi = (7*F1)/12000 - (7*F2)/12000 + (7*F3)/12000 - (7*F4)/12000 - (36799*dphi)/15000 + (5257*dzu1)/6000 - (5257*dzu2)/6000 + (5257*dzu3)/6000 - (5257*dzu4)/6000 - 49*phi + (35*zu1)/2 - (35*zu2)/2 + (35*zu3)/2 - (35*zu4)/2;
 
 
ddzu1 = (751*dphi)/50 - F1/70 + (4506*dtheta)/175 + (751*dzs)/35 - (751*dzu1)/35 + 300*phi + (20000*r1)/7 + (3600*theta)/7 + (3000*zs)/7 - (23000*zu1)/7;
 
 
ddzu2 = (4506*dtheta)/175 - (751*dphi)/50 - F2/70 + (751*dzs)/35 - (751*dzu2)/35 - 300*phi + (20000*r2)/7 + (3600*theta)/7 + (3000*zs)/7 - (23000*zu2)/7;
 
 
ddzu3 = (751*dphi)/50 - F3/70 - (2253*dtheta)/70 + (751*dzs)/35 - (751*dzu3)/35 + 300*phi + (20000*r3)/7 - (4500*theta)/7 + (3000*zs)/7 - (23000*zu3)/7;
 
 
ddzu4 = (751*dzs)/35 - (751*dphi)/50 - (2253*dtheta)/70 - F4/70 - (751*dzu4)/35 - 300*phi + (20000*r4)/7 - (4500*theta)/7 + (3000*zs)/7 - (23000*zu4)/7;
end

== matlab function FULL_CAR_SIM/Full Car Model FLC/MATLAB Function ==
  data: dzs input; zs input; dtheta input; ddzs output; theta input; dphi input; phi input; dzu1 input; zu1 input; dzu2 input; zu2 input; dzu3 input; zu3 input; dzu4 input; zu4 input; F1 input; F2 input; F3 input; F4 input; r1 input; r2 input; ddtheta output; ddphi output; ddzu1 output; ddzu2 output; ddzu3 output; ddzu4 output; r3 input; r4 input
function [ddzs, ddtheta, ddphi, ddzu1, ddzu2, ddzu3, ddzu4] = suspension_dynamics(dzs, zs, dtheta, theta, dphi, phi, dzu1, zu1, dzu2, zu2,  dzu3, zu3, dzu4, zu4, F1, F2, F3, F4,r1, r2, r3, r4)

ddzs = F1/1000 + F2/1000 + F3/1000 + F4/1000 + (2253*dtheta)/2500 - (751*dzs)/125 + (751*dzu1)/500 + (751*dzu2)/500 + (751*dzu3)/500 + (751*dzu4)/500 + 18*theta - 120*zs + 30*zu1 + 30*zu2 + 30*zu3 + 30*zu4;
 
 
ddtheta = F1/1000 + F2/1000 - F3/800 - F4/800 - (92373*dtheta)/10000 + (751*dzs)/1000 + (751*dzu1)/500 + (751*dzu2)/500 - (751*dzu3)/400 - (751*dzu4)/400 - (369*theta)/2 + 15*zs + 30*zu1 + 30*zu2 - (75*zu3)/2 - (75*zu4)/2;
 
 
ddphi = (7*F1)/12000 - (7*F2)/12000 + (7*F3)/12000 - (7*F4)/12000 - (36799*dphi)/15000 + (5257*dzu1)/6000 - (5257*dzu2)/6000 + (5257*dzu3)/6000 - (5257*dzu4)/6000 - 49*phi + (35*zu1)/2 - (35*zu2)/2 + (35*zu3)/2 - (35*zu4)/2;
 
 
ddzu1 = (751*dphi)/50 - F1/70 + (4506*dtheta)/175 + (751*dzs)/35 - (751*dzu1)/35 + 300*phi + (20000*r1)/7 + (3600*theta)/7 + (3000*zs)/7 - (23000*zu1)/7;
 
 
ddzu2 = (4506*dtheta)/175 - (751*dphi)/50 - F2/70 + (751*dzs)/35 - (751*dzu2)/35 - 300*phi + (20000*r2)/7 + (3600*theta)/7 + (3000*zs)/7 - (23000*zu2)/7;
 
 
ddzu3 = (751*dphi)/50 - F3/70 - (2253*dtheta)/70 + (751*dzs)/35 - (751*dzu3)/35 + 300*phi + (20000*r3)/7 - (4500*theta)/7 + (3000*zs)/7 - (23000*zu3)/7;
 
 
ddzu4 = (751*dzs)/35 - (751*dphi)/50 - (2253*dtheta)/70 - F4/70 - (751*dzu4)/35 - 300*phi + (20000*r4)/7 - (4500*theta)/7 + (3000*zs)/7 - (23000*zu4)/7;
end
